simulink model "Porsche930Turbo_Model_V0"  (R2025b)
settings: Solver=ode3  StartTime=0.0  StopTime=1800  FixedStep=0.005  MaxStep=0.01  RelTol=1e-3
values from neighbouring files (symbols this model uses):
  a_front = (1 - CoG_front) * wb    (= 1.32912)    [Main.m]
  af = 1.77    [Main.m]
  bsfc = 395    [Main.m]
  cd = 0.39    [Main.m]
  crr = 0.015    [Main.m]
  distance_imola = s_track    [Main.m]
  eta_gb = 0.95    [Main.m]
  gear_numbers = [1, 2, 3, 4]    [Main.m]
  gear_ratios = [2.25, 1.30, 0.89, 0.625]    [Main.m]
  gear_shift_tbl = [1, 2, 3, 4]    [Main.m]
  grade_imola = grade_track    [Main.m]
  kt = 1.65    [Main.m]
  m_eq = mg + (J_wheels / rw^2) + (J_drivetrain * i_avg^2 / rw^2)    [Main.m]
  mg = mc + (mh * np) + mp_hybrid    (= 1492.5)    [Main.m]
  mu_road = 0.9    [Main.m]
  n_ice = 0:dn:nd    [Main.m]
  ne_em = 0:dn:nemax_em    [Main.m]
  nparallel = 2    [Main.m]
  nseries = 96    [Main.m]
  rho_fuel = 0.75    [Main.m]
  ro = 1.204    [Main.m]
  rt = 4.222    [Main.m]
  rw = (dw * 25.4 / 2 + wt * art / 100) * 1e-3    (= 0.31345)    [Main.m]
  t_ice = zeros(size(n_ice))    [Main.m]
  t_roma_san_basilio = [0 1 2 3 4 5 6 7 8 9 10 11 ... (522 elements, 522x1)]    [ECE_EUDC_Artemis_Bologna_Roma_WLTC_EE_bus.mat]
  tau_turbo = 0.6    [Main.m]
  te_em = zeros(size(ne_em))    [Main.m]
  te_em_peak = zeros(size(ne_em))    [Main.m]
  temax_em = 230    [Main.m]
  tmax_ice = 412    [Main.m]
  track_length = 4909    [Main.m]
  v_cutoff_bp = [0, 0.5, 1.4, 50]    [Main.m]
  v_cutoff_tbl = [0, 0,   1,   1 ]    [Main.m]
  v_ref_imola = v_track_ms    [Main.m]
  v_shift_bp = [0, 18, 33, 48]    [Main.m]
  v_shift_bp_EMODE = [0, 5, 22, 35]    [Main.m]
  vkm_roma_san_basilio = [28.8 30.9 32.4 34.2 35.3 35.6 34.8 33.8 32.2 30.5 29.1 27.9 ... (522 elements, 522x1)]    [ECE_EUDC_Artemis_Bologna_Roma_WLTC_EE_bus.mat]
  wb = 2.272    [Main.m]
undefined symbols (not defined in the file or in its folder): SoC_Per
libraries: simulink x58
(part 4 of 5)

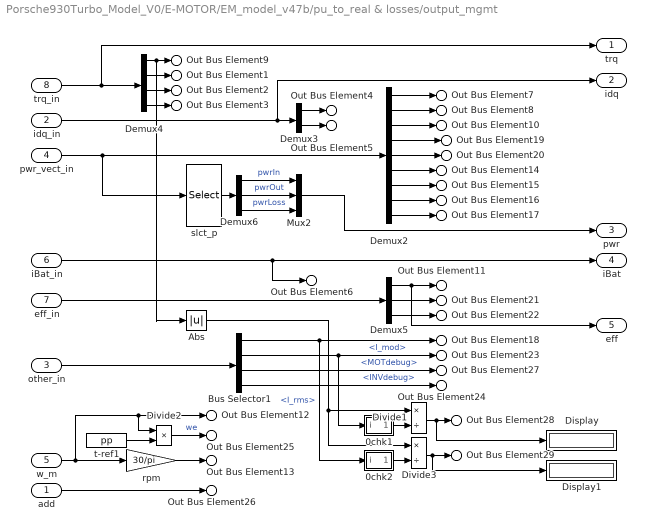
== system Porsche930Turbo_Model_V0/E-MOTOR/EM_model_v47b/pu_to_real & losses/output_mgmt ==
  add : Inport
  idq_in : Inport  Port=2
  other_in : Inport  Port=3
  pwr_vect_in : Inport  Port=4
  w_m : Inport  Port=5
  iBat_in : Inport  Port=6
  eff_in : Inport  Port=7
  trq_in : Inport  Port=8
  0chk1 : Subsystem
      mask Display: disp('0chk')
  0chk2 : Subsystem
      mask Display: disp('0chk')
  Abs : Abs  SaturateOnIntegerOverflow=off
  Bus Selector1 : BusSelector  OutputSignals=I_rms,I_mod,MOTdebug,INVdebug
  Demux2 : Demux  Outputs=9
  Demux3 : Demux  Outputs=2
  Demux4 : Demux
  Demux5 : Demux  Outputs=3
  Demux6 : Demux  Outputs=3
  Display : Display
  Display1 : Display
  Divide1 : Product  Inputs=*/
  Divide2 : Product  Inputs=**
  Divide3 : Product  Inputs=*/
  Mux2 : Mux  Inputs=3
  rpm : Gain  Gain=30/pi  OutDataTypeStr=double
  slct_p : Selector  InputPortWidth=9  IndexOptions=Index vector (dialog)  Indices=[1 2 3]  OutputSizes=1
  t-ref1 : Constant  Value=pp
  trq : Outport
  idq : Outport  Port=2
  pwr : Outport  Port=3
  iBat : Outport  Port=4
  eff : Outport  Port=5
  Out Bus Element9 : Outport  Port=6  PortName=oBus  Element=trqOut
  Out Bus Element1 : Outport  Port=6  PortName=oBus  Element=trqRef
  Out Bus Element2 : Outport  Port=6  PortName=oBus  Element=trqMax
  Out Bus Element3 : Outport  Port=6  PortName=oBus  Element=trqMin
  Out Bus Element4 : Outport  Port=6  PortName=oBus  Element=id
  Out Bus Element5 : Outport  Port=6  PortName=oBus  Element=iq
  Out Bus Element6 : Outport  Port=6  PortName=oBus  Element=iBat
  Out Bus Element18 : Outport  Port=6  PortName=oBus  Element=Irms
  Out Bus Element23 : Outport  Port=6  PortName=oBus  Element=Imod
  Out Bus Element7 : Outport  Port=6  PortName=oBus  Element=pwrIn
  Out Bus Element8 : Outport  Port=6  PortName=oBus  Element=pwrOut
  Out Bus Element10 : Outport  Port=6  PortName=oBus  Element=pwrLoss
  Out Bus Element11 : Outport  Port=6  PortName=oBus  Element=effTot
  Out Bus Element14 : Outport  Port=6  PortName=oBus  Element=pwrOut_Max
  Out Bus Element15 : Outport  Port=6  PortName=oBus  Element=pwrOut_Min
  Out Bus Element16 : Outport  Port=6  PortName=oBus  Element=pwrIn_Max
  Out Bus Element17 : Outport  Port=6  PortName=oBus  Element=pwrIn_Min
  Out Bus Element19 : Outport  Port=6  PortName=oBus  Element=motLosses
  Out Bus Element20 : Outport  Port=6  PortName=oBus  Element=invLosses
  Out Bus Element21 : Outport  Port=6  PortName=oBus  Element=effMot
  Out Bus Element22 : Outport  Port=6  PortName=oBus  Element=effInv
  Out Bus Element28 : Outport  Port=6  PortName=oBus  Element=Kt
  Out Bus Element29 : Outport  Port=6  PortName=oBus  Element=Kt_rms
  Out Bus Element12 : Outport  Port=6  PortName=oBus  Element=w_mec_rads
  Out Bus Element13 : Outport  Port=6  PortName=oBus  Element=w_mec_rpm
  Out Bus Element25 : Outport  Port=6  PortName=oBus  Element=w_ele_rads
  Out Bus Element26 : Outport  Port=6  PortName=oBus  Element=additional
  Out Bus Element24 : Outport  Port=6  PortName=oBus  Element=INVdebug
  Out Bus Element27 : Outport  Port=6  PortName=oBus  Element=MOTdebug
  wires:
  Demux4/1 -> Abs/1, Out Bus Element9/1
  Demux3/1 -> Out Bus Element4/1
  eff_in/1 -> Demux5/1
  Bus Selector1/4 -> Out Bus Element24/1  "<INVdebug>"
  Demux2/6 -> Out Bus Element14/1
  Bus Selector1/2 -> Out Bus Element23/1, 0chk1/1(i)  "<I_mod>"
  Demux2/1 -> Out Bus Element7/1
  Demux4/3 -> Out Bus Element2/1
  Demux3/2 -> Out Bus Element5/1
  Demux2/2 -> Out Bus Element8/1
  Demux5/3 -> Out Bus Element22/1
  Demux2/7 -> Out Bus Element15/1
  Demux2/9 -> Out Bus Element17/1
  Demux4/4 -> Out Bus Element3/1
  Demux4/2 -> Out Bus Element1/1
  Demux2/4 -> Out Bus Element19/1
  Demux2/3 -> Out Bus Element10/1
  Demux2/5 -> Out Bus Element20/1
  Demux5/2 -> Out Bus Element21/1
  Demux2/8 -> Out Bus Element16/1
  Bus Selector1/1 -> Out Bus Element18/1, 0chk2/1(i)  "<I_rms>"
  rpm/1 -> Out Bus Element13/1
  w_m/1 -> Divide2/1, Out Bus Element12/1, rpm/1
  other_in/1 -> Bus Selector1/1
  trq_in/1 -> trq/1, Demux4/1
  slct_p/1 -> Demux6/1
  idq_in/1 -> idq/1, Demux3/1
  pwr_vect_in/1 -> Demux2/1, slct_p/1
  Demux6/3 -> Mux2/3  "pwrLoss"
  Demux6/1 -> Mux2/1  "pwrIn"
  iBat_in/1 -> Out Bus Element6/1, iBat/1
  Mux2/1 -> pwr/1
  Demux5/1 -> Out Bus Element11/1, eff/1
  Demux6/2 -> Mux2/2  "pwrOut"
  t-ref1/1 -> Divide2/2
  Divide2/1 -> Out Bus Element25/1  "we"
  add/1 -> Out Bus Element26/1
  Bus Selector1/3 -> Out Bus Element27/1  "<MOTdebug>"
  Divide1/1 -> Display/1, Out Bus Element28/1
  Divide3/1 -> Out Bus Element29/1, Display1/1
  0chk2/1(o) -> Divide3/2
  0chk1/1(o) -> Divide1/2
  Abs/1 -> Divide3/1, Divide1/1

== system Porsche930Turbo_Model_V0/E-MOTOR/EM_model_v47b/pu_to_real & losses/pwr_calc ==
  pwr_loss : Inport
  w_m : Inport  Port=2
  trq : Inport  Port=3
  Demux4 : Demux  Outputs=2
  Divide2 : Product  Inputs=**
  Divide3 : Product  Inputs=**
  MaxMin : Selector  InputPortWidth=4  IndexOptions=Index vector (dialog)  Indices=[3 4]  OutputSizes=1
  Mux5 : Mux  Inputs=7
  Sum1 : Sum
  Sum2 : Sum
  Sum3 : Sum  Inputs=+
  trq_out : Selector  InputPortWidth=4  IndexOptions=Index vector (dialog)  Indices=1  OutputSizes=1
  pwr_vect : Outport
  pwrIN : Outport  Port=2
  wires:
  w_m/1 -> Divide3/1, Divide2/1
  trq_out/1 -> Divide2/2
  trq/1 -> trq_out/1, MaxMin/1
  MaxMin/1 -> Divide3/2
  Divide3/1 -> Sum2/1, Mux5/6  "pwrMaxOUT"
  Sum2/1 -> Mux5/7  "pwrMaxIN"
  Sum3/1 -> Mux5/3, Sum2/2, Sum1/1  "pwrLOSS"
  Divide2/1 -> Sum1/2, Mux5/2  "pwrOUT"
  Sum1/1 -> pwrIN/1, Mux5/1  "pwrIN"
  Mux5/1 -> pwr_vect/1
  pwr_loss/1 -> Demux4/1, Sum3/1
  Demux4/1 -> Mux5/4  "mot_loss"
  Demux4/2 -> Mux5/5  "inv_loss"

== system Porsche930Turbo_Model_V0/E-MOTOR/EM_model_v47b/pu_to_real & losses/trq_derating_TBD ==
  note: recalculation of Irms
      | saturated, mainly for
      | verification
  note: linear idq is increased
      | by "saturation coeff"
  note: outputs Irms saturated
      | given the torque input
  note: VERIFICATION
  idq : Inport
  idq_pu : Inport  Port=2
  trq_pu : Inport  Port=3
  trqIn : Inport  Port=4
  0chk : Subsystem
      mask Display: disp('0chk')
  0chk1 : Subsystem
      mask Display: disp('0chk')
  0chk2 : Subsystem
      mask Display: disp('0chk')
  Abs1 : Abs  SaturateOnIntegerOverflow=off
  DQmodule : Subsystem
      mask Display: disp('DQmod')
  DQmodule1 : Subsystem
      mask Display: disp('DQmod')
  DQmodule2 : Subsystem
      mask Display: disp('DQmod')
  Divide1 : Product  Inputs=**
  Divide2 : Product  Inputs=*/
  Divide4 : Product  Inputs=/*
  Divide5 : Product  Inputs=/*
  peak2rms : Subsystem
      mask Display: disp('pk2rms')
  peak2rms1 : Subsystem
      mask Display: disp('pk2rms')
  peak2rms2 : Subsystem
      mask Display: disp('pk2rms')
  sc{1..3,5,8} (5 alike) : Scope  NumInputPorts=2
      sc1 settings: DataLoggingSaveFormat=Array
      sc2 settings: DataLoggingVariableName=ScopeData5  DataLoggingSaveFormat=Array
      sc3 settings: DataLoggingVariableName=ScopeData5  DataLoggingSaveFormat=Array
      sc5 settings: DataLoggingVariableName=ScopeData9  DataLoggingSaveFormat=Array
      sc8 settings: DataLoggingVariableName=ScopeData13  DataLoggingSaveFormat=Array
  sc6 : Scope  NumInputPorts=3
      settings: DataLoggingVariableName=ScopeData10  DataLoggingSaveFormat=Array
  trq vs curr : Lookup_n-D  NumberOfTableDimensions=1  BreakpointsForDimension1=[0 0.5 0.75 1 1.4 1.8 2.5 3]  BeginIndexSearchUsingPreviousIndexResult=on  Table=[0 0.5 0.75 1 1.5 2 3 4]  InternalRulePriority=Speed  RndMeth=Simplest
  trq_out : Selector  InputPortWidth=4  IndexOptions=Index vector (dialog)  Indices=1  OutputSizes=1
  trq_outPU : Selector  InputPortWidth=4  IndexOptions=Index vector (dialog)  Indices=1  OutputSizes=1
  idq_sat : Outport
  wires:
  trqIn/1 -> trq_out/1
  trq_out/1 -> Divide5/2, Divide4/2
  peak2rms1/1(o) -> 0chk1/1(i)
  trq vs curr/1 -> sc2/2, sc6/2, Divide2/1  "Irms"
  idq/1 -> Divide1/1, DQmodule1/1(i), sc1/1
  Divide2/1 -> sc3/2, Divide1/2
  Divide1/1 -> DQmodule2/1(i), idq_sat/1
  peak2rms2/1(o) -> 0chk2/1(i), sc6/1
  Divide4/1 -> sc8/2
  Divide5/1 -> sc8/1
  DQmodule1/1(mod) -> peak2rms1/1(i), sc5/1, sc1/2
  0chk1/1(o) -> sc2/1, Divide4/1, sc6/3
  0chk2/1(o) -> Divide5/1
  idq_pu/1 -> DQmodule/1(i)
  trq_pu/1 -> trq_outPU/1
  trq_outPU/1 -> Abs1/1
  peak2rms/1(o) -> 0chk/1(i)
  DQmodule/1(mod) -> peak2rms/1(i)
  0chk/1(o) -> sc3/1, Divide2/2
  Abs1/1 -> trq vs curr/1
  DQmodule2/1(mod) -> peak2rms2/1(i), sc5/2

== system Porsche930Turbo_Model_V0/E-MOTOR/EM_model_v47b/real_to_pu & param/input_iLim ==
  i : Inport
  Display1 : Display
  Multiport Switch1 : MultiPortSwitch  SaturateOnIntegerOverflow=off  InputSameDT=off
  t-ref2 : Constant  Value=overl
  t-ref7 : Constant  Value=i_lim
  t-ref8 : Constant
  iLim : Outport
  wires:
  i/1 -> Multiport Switch1/4  "from port"
  Multiport Switch1/1 -> iLim/1
  t-ref2/1 -> Display1/1, Multiport Switch1/1
  t-ref7/1 -> Multiport Switch1/3  "static"
  t-ref8/1 -> Multiport Switch1/2  "no overload"

== system Porsche930Turbo_Model_V0/E-MOTOR/EM_model_v47b/real_to_pu & param/input_rs ==
  i : Inport
  Display6 : Display
  Multiport Switch1 : MultiPortSwitch  SaturateOnIntegerOverflow=off  InputSameDT=off
  n 1 : Constant  Value=rs
  n 2 : Constant  Value=1e-6
  t-ref1 : Constant  Value=RsSlct
  rs : Outport
  wires:
  i/1 -> Multiport Switch1/4  "from port"
  Multiport Switch1/1 -> rs/1
  t-ref1/1 -> Multiport Switch1/1, Display6/1
  n 2/1 -> Multiport Switch1/2  "no stator res"
  n 1/1 -> Multiport Switch1/3  "static"

== system Porsche930Turbo_Model_V0/E-MOTOR/EM_model_v47b/real_to_pu & param/input_spd ==
  i : Inport
  Display1 : Display
  Multiport Switch1 : MultiPortSwitch  Inputs=2  SaturateOnIntegerOverflow=off  InputSameDT=off
  rad/s : Gain  Gain=pi/30  OutDataTypeStr=double
  t-ref : Constant  Value=spdIn
  rads : Outport
  wires:
  rad/s/1 -> Multiport Switch1/2
  i/1 -> rad/s/1, Multiport Switch1/3
  Multiport Switch1/1 -> rads/1
  t-ref/1 -> Multiport Switch1/1, Display1/1

== system Porsche930Turbo_Model_V0/E-MOTOR/EM_model_v47b/real_to_pu & param/spd_0chk ==
  i : Inport
  Abs : Abs  SaturateOnIntegerOverflow=off
  MinMax1 : MinMax  Function=max  Inputs=2
  Switch3 : Switch  SaturateOnIntegerOverflow=off  InputSameDT=off
  V1 : Constant  Value=-1
  V3 : Constant
  n 2 : Constant  Value=1e-4
  x1 : Product  Inputs=**
  o : Outport
  wires:
  n 2/1 -> MinMax1/2
  Switch3/1 -> x1/1
  i/1 -> Switch3/2, Abs/1
  Abs/1 -> MinMax1/1
  x1/1 -> o/1
  V3/1 -> Switch3/1
  V1/1 -> Switch3/3
  MinMax1/1 -> x1/2

== system Porsche930Turbo_Model_V0/E-MOTOR/EM_model_v47b/real_to_pu & param/trq_0chk ==
  i : Inport
  Abs1 : Abs  SaturateOnIntegerOverflow=off
  MinMax1 : MinMax  Function=max  Inputs=2
  Relational Operator1 : RelationalOperator  Operator=<  OutDataTypeStr=boolean  InputSameDT=off
  Switch1 : Switch  SaturateOnIntegerOverflow=off  InputSameDT=off
  V2 : Constant  Value=-1
  V4 : Constant
  range : Constant  Value=0.01
  x1 : Product  Inputs=**
  ctrl0 : Outport
  "o " : Outport  Port=2
  wires:
  x1/1 -> "o "/1
  MinMax1/1 -> x1/2
  V2/1 -> Switch1/3
  V4/1 -> Switch1/1
  Abs1/1 -> Relational Operator1/1, MinMax1/1
  i/1 -> Switch1/2, Abs1/1
  Switch1/1 -> x1/1
  range/1 -> Relational Operator1/2, MinMax1/2
  Relational Operator1/1 -> ctrl0/1

== system Porsche930Turbo_Model_V0/Battery Pack/Subsystem/Thermal Model/Subsystem/Subsystem ==
  R1 [°C/W] : Inport
  R2 [°C/W] : Inport  Port=2
  R3 [°C/W] : Inport  Port=3
  C1 [J/°C] : Inport  Port=4
  C2 [J/°C] : Inport  Port=5
  Sum : Sum
  Tau : Sum  Inputs=+++
  Tau1 : Product
  Tau12 : Product
  Tau2 : Product
  tau [J/W] : Outport
  tau1 [J/W] : Outport  Port=2
  tau2 [J/W] : Outport  Port=3
  tau12 [J/W] : Outport  Port=4
  wires:
  Tau1/1 -> tau1 [J/W]/1, Tau/1
  Sum/1 -> Tau12/1, Tau2/1
  Tau2/1 -> Tau/2, tau2 [J/W]/1
  C2 [J/°C]/1 -> Tau2/2
  Tau12/1 -> Tau/3, tau12 [J/W]/1
  Tau/1 -> tau [J/W]/1
  C1 [J/°C]/1 -> Tau1/2, Tau12/2
  R1 [°C/W]/1 -> Tau1/1
  R3 [°C/W]/1 -> Sum/2
  R2 [°C/W]/1 -> Sum/1

== system Porsche930Turbo_Model_V0/Battery Pack/Subsystem/Thermal Model/Subsystem1/Subsystem ==
  R1 [°C/W] : Inport
  R3 [°C/W] : Inport  Port=2
  C1 [J/°C] : Inport  Port=3
  Product : Product
  Sum : Sum
  tau [J/W] : Outport
  wires:
  R3 [°C/W]/1 -> Sum/2
  R1 [°C/W]/1 -> Sum/1
  Sum/1 -> Product/1
  C1 [J/°C]/1 -> Product/2
  Product/1 -> tau [J/W]/1

== system Porsche930Turbo_Model_V0/E-MOTOR/EM_model_v47b/Motor_Model/blockB/module MTV ==
  i : Inport
  Add : Sum
  Demux2 : Demux  Outputs=2
  Product : Product
  Product1 : Product
  Sqrt : Sqrt
  mod : Outport
  wires:
  Demux2/1 -> Product/2, Product/1
  Sqrt/1 -> mod/1
  Product/1 -> Add/1
  Demux2/2 -> Product1/1, Product1/2
  Add/1 -> Sqrt/1
  Product1/1 -> Add/2
  i/1 -> Demux2/1

== system Porsche930Turbo_Model_V0/E-MOTOR/EM_model_v47b/Motor_Model/blockB/module TF ==
  i : Inport
  Add : Sum
  Demux2 : Demux  Outputs=2
  Product : Product
  Product1 : Product
  Sqrt : Sqrt
  mod : Outport
  wires:
  Demux2/1 -> Product/2, Product/1
  Sqrt/1 -> mod/1
  Product/1 -> Add/1
  Demux2/2 -> Product1/1, Product1/2
  Add/1 -> Sqrt/1
  Product1/1 -> Add/2
  i/1 -> Demux2/1

== system Porsche930Turbo_Model_V0/E-MOTOR/EM_model_v47b/Motor_Model/blockC/0chk ==
  i : Inport
  Abs : Abs  SaturateOnIntegerOverflow=off
  MinMax1 : MinMax  Function=max  Inputs=2
  Switch3 : Switch  SaturateOnIntegerOverflow=off  InputSameDT=off
  V1 : Constant  Value=-1
  V3 : Constant
  n 2 : Constant  Value=1e-6
  x1 : Product  Inputs=**
  o : Outport
  wires:
  n 2/1 -> MinMax1/2
  Switch3/1 -> x1/1
  i/1 -> Switch3/2, Abs/1
  Abs/1 -> MinMax1/1
  x1/1 -> o/1
  V3/1 -> Switch3/1
  V1/1 -> Switch3/3
  MinMax1/1 -> x1/2

== system Porsche930Turbo_Model_V0/E-MOTOR/EM_model_v47b/Motor_Model/blockD/idq_max_MTC-I0 ==
  trq : Inport
  I0 : Inport  Port=2
  "0 " : Constant  Value=0
  Compare To Constant3 : simulink/Logic and Bit Operations/Compare To Constant  relop===  const=1  OutDataTypeStr=boolean
  Constant4 : Constant  Value=r
  Divide2 : Product  Inputs=**
  Gain1 : Gain  Gain=-1
  Mux2 : Mux  Inputs=2
  Mux5 : Mux  Inputs=2
  Switch7 : Switch  Criteria=u2 > Threshold  SaturateOnIntegerOverflow=off  InputSameDT=off
  id_mtcMax : Subsystem
  iq_mtcMax : Subsystem
  sign : Subsystem
  idq_mtcMaxPos : Outport
  idq_mtcMaxNeg : Outport  Port=2
  wires:
  Switch7/1 -> iq_mtcMax/2(id), Mux5/1, Mux2/1
  "0 "/1 -> Switch7/1
  I0/1 -> iq_mtcMax/1(IO), id_mtcMax/1(I0)
  sign/1(o) -> Divide2/2
  trq/1 -> sign/1(i)
  Constant4/1 -> Compare To Constant3/1
  Compare To Constant3/1 -> Switch7/2
  iq_mtcMax/1(iq) -> Divide2/1
  id_mtcMax/1(id_MTC) -> Switch7/3
  Divide2/1 -> Gain1/1, Mux5/2
  Mux5/1 -> idq_mtcMaxPos/1
  Gain1/1 -> Mux2/2
  Mux2/1 -> idq_mtcMaxNeg/1

== system Porsche930Turbo_Model_V0/E-MOTOR/EM_model_v47b/Motor_Model/blockD/idq_max_MTV-I0 ==
  b : Inport
  theta : Inport  Port=2
  trq : Inport  Port=3
  I0 : Inport  Port=4
  Gain2 : Gain  Gain=-1
  Mux1 : Mux  Inputs=2
  Mux3 : Mux  Inputs=2
  a : Constant  Value=a
  intersections_neg : MATLAB Function  TreatAsAtomicUnit=on
  intersections_pos : MATLAB Function  TreatAsAtomicUnit=on
  r 1 : Constant  Value=r
  sc1 : Scope  NumInputPorts=2
      settings: DataLoggingVariableName=ScopeData5  DataLoggingSaveFormat=Array
  sc2 : Scope  NumInputPorts=2
      settings: DataLoggingVariableName=ScopeData4  DataLoggingSaveFormat=Array
  flg_maxSpd : Outport
  idq_mtvMaxPos : Outport  Port=2
  idq_mtvMaxNeg : Outport  Port=3
  wires:
  a/1 -> intersections_neg/1(a), intersections_pos/1(a)
  r 1/1 -> intersections_neg/2(r), intersections_pos/2(r)
  intersections_pos/1(id) -> Mux3/1  "id_mtv"
  intersections_pos/2(iq) -> Mux3/2  "iq_mtv"
  intersections_pos/3(discr) -> sc2/2, flg_maxSpd/1
  b/1 -> intersections_neg/3(b), intersections_pos/3(b)
  I0/1 -> intersections_neg/4(I0), intersections_pos/4(I0)
  theta/1 -> intersections_neg/5(theta), intersections_pos/5(theta)
  trq/1 -> Gain2/1, intersections_pos/6(t)
  Gain2/1 -> intersections_neg/6(t)
  intersections_neg/1(id) -> Mux1/1  "id_mtv"
  intersections_neg/2(iq) -> Mux1/2  "iq_mtv"
  Mux3/1 -> sc2/1, idq_mtvMaxPos/1
  Mux1/1 -> sc1/1, idq_mtvMaxNeg/1
  intersections_neg/3(discr) -> sc1/2

== system Porsche930Turbo_Model_V0/E-MOTOR/EM_model_v47b/Motor_Model/blockD/iso controller ==
  id_b_pos : Inport
  id_b_neg : Inport  Port=2
  id_MTC : Inport  Port=3
  Compare To Constant : simulink/Logic and Bit Operations/Compare To Constant  relop=>  const=1  OutDataTypeStr=boolean
  Compare To Constant1 : simulink/Logic and Bit Operations/Compare To Constant  relop=~=  const=0  OutDataTypeStr=boolean
  Compare To Constant2 : simulink/Logic and Bit Operations/Compare To Constant  relop=~=  const=0  OutDataTypeStr=boolean
  Compare To Constant3 : simulink/Logic and Bit Operations/Compare To Constant  relop===  const=1  OutDataTypeStr=boolean
  Constant : Constant  Value=r
  Constant4 : Constant  Value=r
  Constant5 : Constant  Value=0
  Logical Operator : Logic  AllPortsSameDT=off  OutDataTypeStr=boolean
  Logical Operator1 : Logic  AllPortsSameDT=off  OutDataTypeStr=boolean
  Relational Operator1 : RelationalOperator  Operator=<=  OutDataTypeStr=boolean  InputSameDT=off
  Relational Operator3 : RelationalOperator  Operator=<=  OutDataTypeStr=boolean  InputSameDT=off
  Switch1 : Switch  Criteria=u2 > Threshold  SaturateOnIntegerOverflow=off  InputSameDT=off
  Switch2 : Switch  Criteria=u2 > Threshold  SaturateOnIntegerOverflow=off  InputSameDT=off
  Switch3 : Switch  Criteria=u2 > Threshold  SaturateOnIntegerOverflow=off  InputSameDT=off
  scope2 : Scope  NumInputPorts=2
      settings: DataLoggingSaveFormat=Array
  cont_pos : Outport
  cont_neg : Outport  Port=2
  wires:
  Constant/1 -> Compare To Constant/1
  Switch2/1 -> scope2/1, cont_pos/1
  Compare To Constant/1 -> Switch1/2, Switch2/2
  Relational Operator3/1 -> Switch2/3, Logical Operator/1
  Compare To Constant1/1 -> Logical Operator/2
  Logical Operator/1 -> Switch2/1
  id_b_pos/1 -> Compare To Constant1/1, Relational Operator3/1
  Switch3/1 -> Relational Operator3/2, Relational Operator1/2
  id_MTC/1 -> Switch3/3
  Constant4/1 -> Compare To Constant3/1
  Compare To Constant3/1 -> Switch3/2
  Constant5/1 -> Switch3/1
  Compare To Constant2/1 -> Logical Operator1/2
  Relational Operator1/1 -> Switch1/3, Logical Operator1/1
  Logical Operator1/1 -> Switch1/1
  id_b_neg/1 -> Compare To Constant2/1, Relational Operator1/1
  Switch1/1 -> scope2/2, cont_neg/1

== system Porsche930Turbo_Model_V0/E-MOTOR/EM_model_v47b/Motor_Model/blockE/module ==
  in : Inport
  Add : Sum
  Demux2 : Demux  Outputs=2
  Product : Product
  Product1 : Product
  Sqrt : Sqrt
  module : Outport
  wires:
  Demux2/1 -> Product/2, Product/1
  Sqrt/1 -> module/1
  Product/1 -> Add/1
  Demux2/2 -> Product1/1, Product1/2
  Add/1 -> Sqrt/1
  Product1/1 -> Add/2
  in/1 -> Demux2/1

== system Porsche930Turbo_Model_V0/E-MOTOR/EM_model_v47b/Motor_Model/limit_rpm/trq calc ==
  idq : Inport
  Add : Sum
  Constant10 : Constant  Value=r1
  Constant11 : Constant  Value=a
  Demux1 : Demux  Outputs=2
  Product3 : Product  Inputs=3
  Product7 : Product
  trq : Outport
  wires:
  idq/1 -> Demux1/1
  Constant10/1 -> Product3/3
  Add/1 -> trq/1
  Demux1/1 -> Product3/1
  Product7/1 -> Add/2
  Product3/1 -> Add/1
  Demux1/2 -> Product7/1, Product3/2
  Constant11/1 -> Product7/2

== system Porsche930Turbo_Model_V0/E-MOTOR/EM_model_v47b/Motor_Model/limits_MaxMin/DQmodule ==
  i : Inport
  Add : Sum
  Demux2 : Demux  Outputs=2
  Product : Product
  Product1 : Product
  Sqrt : Sqrt
  mod : Outport
  wires:
  Demux2/1 -> Product/2, Product/1
  Sqrt/1 -> mod/1
  Product/1 -> Add/1
  Demux2/2 -> Product1/1, Product1/2
  Add/1 -> Sqrt/1
  Product1/1 -> Add/2
  i/1 -> Demux2/1

== system Porsche930Turbo_Model_V0/E-MOTOR/EM_model_v47b/Motor_Model/limits_MaxMin/MTV_sat_low spd ==
  i_lim : Inport
  idq_ref : Inport  Port=2
  mod_chk : Inport  Port=3
  Demux2 : Demux
  Demux6 : Demux  Outputs=2
  MinMax3 : MinMax  Function=max  Inputs=2
  MinMax4 : MinMax  Inputs=2
  MinMax5 : MinMax  Function=max  Inputs=2
  MinMax6 : MinMax  Inputs=2
  Mux14 : Mux  Inputs=2
  SatDyn : simulink/Discontinuities/Saturation Dynamic  OutMin=[]  OutMax=[]  OutDataTypeStr=Inherit: Same as second input  OutDataType=fixdt(1, 16)  OutScaling=2^-10  DoSatur=off
  SatDyn1 : simulink/Discontinuities/Saturation Dynamic  OutMin=[]  OutMax=[]  OutDataTypeStr=Inherit: Same as second input  OutDataType=fixdt(1, 16)  OutScaling=2^-10  DoSatur=off
  Switch12 : Switch  Criteria=u2 > Threshold  SaturateOnIntegerOverflow=off  InputSameDT=off
  idq_sat : Outport
  wires:
  Mux14/1 -> Switch12/1
  Demux6/2 -> SatDyn1/2  "iq"
  mod_chk/1 -> Switch12/2
  Demux6/1 -> SatDyn/2  "id"
  MinMax6/1 -> SatDyn1/3
  MinMax3/1 -> SatDyn/1
  MinMax4/1 -> SatDyn/3
  Demux2/3 -> MinMax3/2, MinMax4/2  "id2"
  Demux2/2 -> MinMax5/1, MinMax6/1  "iq1"
  Demux2/4 -> MinMax6/2, MinMax5/2  "iq2"
  Demux2/1 -> MinMax4/1, MinMax3/1  "id1"
  MinMax5/1 -> SatDyn1/1
  Switch12/1 -> idq_sat/1
  SatDyn1/1 -> Mux14/2
  SatDyn/1 -> Mux14/1
  idq_ref/1 -> Demux6/1, Switch12/3
  i_lim/1 -> Demux2/1

== system Porsche930Turbo_Model_V0/E-MOTOR/EM_model_v47b/Motor_Model/limits_MaxMin/current limits calc ==
  I0 : Inport
  I0_lim : Inport  Port=2
  MTV_lim : Inport  Port=3
  Comp2Const2 : simulink/Logic and Bit Operations/Compare To Constant  relop===  const=0  OutDataTypeStr=boolean
  Comp2Const3 : simulink/Logic and Bit Operations/Compare To Constant  relop===  const=0  OutDataTypeStr=boolean
  DQmodule : Subsystem
      mask Display: disp('DQmod')
  DQmodule1 : Subsystem
      mask Display: disp('DQmod')
  Demux1 : Demux
  Demux4 : Demux
  Logical Operator3 : Logic  Operator=OR  AllPortsSameDT=off  OutDataTypeStr=boolean
  Logical Operator4 : Logic  Operator=OR  AllPortsSameDT=off  OutDataTypeStr=boolean
  Mux{2..3,5..6,8} (5 alike) : Mux  Inputs=2
  Relational Operator1 : RelationalOperator  Operator=>  OutDataTypeStr=boolean  InputSameDT=off
  Relational Operator3 : RelationalOperator  Operator=>  OutDataTypeStr=boolean  InputSameDT=off
  Switch3 : Switch  Criteria=u2 > Threshold  SaturateOnIntegerOverflow=off  InputSameDT=off
  Switch6 : Switch  Criteria=u2 > Threshold  SaturateOnIntegerOverflow=off  InputSameDT=off
  losses4 : Scope  NumInputPorts=2
      settings: DataLoggingVariableName=ScopeData12  DataLoggingSaveFormat=Array
  losses6 : Scope  NumInputPorts=3
      settings: DataLoggingVariableName=ScopeData15  DataLoggingSaveFormat=Array
  i_limit_MaxMin : Outport
  moduleMTV : Outport  Port=2
  wires:
  MTV_lim/1 -> Demux4/1
  Mux3/1 -> [I0_lim2]
  Relational Operator3/1 -> Logical Operator4/1
  Relational Operator1/1 -> Logical Operator3/1
  Demux1/4 -> Mux3/2
  Demux4/4 -> Mux2/2
  Switch3/1 -> Mux8/1
  Demux1/1 -> Mux6/1
  Demux4/1 -> Mux5/1
  Demux1/2 -> Mux6/2
  Mux6/1 -> [I0_lim1]
  Switch6/1 -> Mux8/2
  Comp2Const3/1 -> Logical Operator4/2
  I0/1 -> losses6/3, Relational Operator3/2, Relational Operator1/2
  Mux8/1 -> i_limit_MaxMin/1
  Comp2Const2/1 -> Logical Operator3/2
  Logical Operator3/1 -> Switch3/2, losses4/1
  DQmodule/1(mod) -> losses6/2, moduleMTV/1, Comp2Const3/1, Relational Operator3/1
  Demux1/3 -> Mux3/1
  Mux5/1 -> DQmodule1/1(i), [mtv_lim1]
  Logical Operator4/1 -> Switch6/2, losses4/2
  Demux4/2 -> Mux5/2
  DQmodule1/1(mod) -> Relational Operator1/1, Comp2Const2/1, losses6/1
  I0_lim/1 -> Demux1/1
  Demux4/3 -> Mux2/1
  Mux2/1 -> DQmodule/1(i), [mtv_lim2]
  [I0_lim1] -> Switch3/1
  [I0_lim2] -> Switch6/1
  [mtv_lim1] -> Switch3/3
  [mtv_lim2] -> Switch6/3

== system Porsche930Turbo_Model_V0/E-MOTOR/EM_model_v47b/Motor_Model/limits_MaxMin/iq from trq+idsat ==
  trq : Inport
  Add1 : Sum
  Constant10 : Constant  Value=r1
  Constant4 : Constant  Value=a
  Constant5 : Constant  Value=sat
  Product1 : Product
  Product2 : Product  Inputs=*/
  scope1 : Scope  NumInputPorts=2
      settings: DataLoggingVariableName=ScopeData3  DataLoggingSaveFormat=Array
  iq : Outport
  wires:
  Constant10/1 -> Product1/1
  Constant5/1 -> Product1/2
  Product1/1 -> Add1/1
  Constant4/1 -> Add1/2
  Add1/1 -> Product2/2, scope1/2
  trq/1 -> scope1/1, Product2/1
  Product2/1 -> iq/1

== system Porsche930Turbo_Model_V0/E-MOTOR/EM_model_v47b/Motor_Model/limits_MaxMin/trq calc1 ==
  idq : Inport
  Add : Sum
  Constant10 : Constant  Value=r1
  Constant11 : Constant  Value=a
  Demux1 : Demux  Outputs=2
  Product3 : Product  Inputs=3
  Product7 : Product
  trq : Outport
  wires:
  idq/1 -> Demux1/1
  Constant10/1 -> Product3/3
  Add/1 -> trq/1
  Demux1/1 -> Product3/1
  Product7/1 -> Add/2
  Product3/1 -> Add/1
  Demux1/2 -> Product7/1, Product3/2
  Constant11/1 -> Product7/2

== system Porsche930Turbo_Model_V0/E-MOTOR/EM_model_v47b/Motor_Model/limits_MaxMin/trq calc2 ==
  idq : Inport
  Add : Sum
  Constant10 : Constant  Value=r1
  Constant11 : Constant  Value=a
  Demux1 : Demux  Outputs=2
  Product3 : Product  Inputs=3
  Product7 : Product
  trq : Outport
  wires:
  idq/1 -> Demux1/1
  Constant10/1 -> Product3/3
  Add/1 -> trq/1
  Demux1/1 -> Product3/1
  Product7/1 -> Add/2
  Product3/1 -> Add/1
  Demux1/2 -> Product7/1, Product3/2
  Constant11/1 -> Product7/2

== system Porsche930Turbo_Model_V0/E-MOTOR/EM_model_v47b/Motor_Model/limits_MaxMin/trq calc3 ==
  idq : Inport
  Add : Sum
  Constant10 : Constant  Value=r1
  Constant11 : Constant  Value=a
  Demux1 : Demux  Outputs=2
  Product3 : Product  Inputs=3
  Product7 : Product
  trq : Outport
  wires:
  idq/1 -> Demux1/1
  Constant10/1 -> Product3/3
  Add/1 -> trq/1
  Demux1/1 -> Product3/1
  Product7/1 -> Add/2
  Product3/1 -> Add/1
  Demux1/2 -> Product7/1, Product3/2
  Constant11/1 -> Product7/2

== system Porsche930Turbo_Model_V0/E-MOTOR/EM_model_v47b/pu_to_real & losses/Additional Calc/0chk ==
  i : Inport
  Abs : Abs  SaturateOnIntegerOverflow=off
  MinMax1 : MinMax  Function=max  Inputs=2
  Switch3 : Switch  SaturateOnIntegerOverflow=off  InputSameDT=off
  V1 : Constant  Value=-1
  V3 : Constant
  n 2 : Constant  Value=1e-8
  x1 : Product  Inputs=**
  o : Outport
  wires:
  n 2/1 -> MinMax1/2
  Switch3/1 -> x1/1
  i/1 -> Switch3/2, Abs/1
  Abs/1 -> MinMax1/1
  x1/1 -> o/1
  V3/1 -> Switch3/1
  V1/1 -> Switch3/3
  MinMax1/1 -> x1/2

== system Porsche930Turbo_Model_V0/E-MOTOR/EM_model_v47b/pu_to_real & losses/Additional Calc/0chk1 ==
  i : Inport
  Abs : Abs  SaturateOnIntegerOverflow=off
  MinMax1 : MinMax  Function=max  Inputs=2
  Switch3 : Switch  SaturateOnIntegerOverflow=off  InputSameDT=off
  V1 : Constant  Value=-1
  V3 : Constant
  n 2 : Constant  Value=1e-8
  x1 : Product  Inputs=**
  o : Outport
  wires:
  n 2/1 -> MinMax1/2
  Switch3/1 -> x1/1
  i/1 -> Switch3/2, Abs/1
  Abs/1 -> MinMax1/1
  x1/1 -> o/1
  V3/1 -> Switch3/1
  V1/1 -> Switch3/3
  MinMax1/1 -> x1/2

== system Porsche930Turbo_Model_V0/E-MOTOR/EM_model_v47b/pu_to_real & losses/Additional Calc/DQmodule ==
  i : Inport
  Add : Sum
  Demux2 : Demux  Outputs=2
  Product : Product
  Product1 : Product
  Sqrt : Sqrt
  mod : Outport
  wires:
  Demux2/1 -> Product/2, Product/1
  Sqrt/1 -> mod/1
  Product/1 -> Add/1
  Demux2/2 -> Product1/1, Product1/2
  Add/1 -> Sqrt/1
  Product1/1 -> Add/2
  i/1 -> Demux2/1

== system Porsche930Turbo_Model_V0/E-MOTOR/EM_model_v47b/pu_to_real & losses/Additional Calc/DQmodule1 ==
  i : Inport
  Add : Sum
  Demux2 : Demux  Outputs=2
  Product : Product
  Product1 : Product
  Sqrt : Sqrt
  mod : Outport
  wires:
  Demux2/1 -> Product/2, Product/1
  Sqrt/1 -> mod/1
  Product/1 -> Add/1
  Demux2/2 -> Product1/1, Product1/2
  Add/1 -> Sqrt/1
  Product1/1 -> Add/2
  i/1 -> Demux2/1

== system Porsche930Turbo_Model_V0/E-MOTOR/EM_model_v47b/pu_to_real & losses/Additional Calc/Torque ==
  fiPM : Inport
  idq : Inport  Port=2
  (Ld-Lq)idiq : Product  Inputs=3
  Constant4 : Constant  Value=Lq
  Constant5 : Constant  Value=(3/2)*pp
  Constant6 : Constant  Value=Ld
  Demux2 : Demux  Outputs=2
  Product7 : Product
  Subtract4 : Sum  Inputs=+-
  Subtract5 : Sum
  fiPM*iq : Product
  EM torque : Outport
  wires:
  idq/1 -> Demux2/1
  fiPM/1 -> fiPM*iq/2
  Product7/1 -> EM torque/1  "EM torque"
  Subtract4/1 -> (Ld-Lq)idiq/1  "Ld-Lq"
  Constant6/1 -> Subtract4/1
  Demux2/1 -> (Ld-Lq)idiq/3  "id"
  Constant5/1 -> Product7/1
  Demux2/2 -> fiPM*iq/1, (Ld-Lq)idiq/2  "iq"
  Constant4/1 -> Subtract4/2
  fiPM*iq/1 -> Subtract5/1
  Subtract5/1 -> Product7/2
  (Ld-Lq)idiq/1 -> Subtract5/2

== system Porsche930Turbo_Model_V0/E-MOTOR/EM_model_v47b/pu_to_real & losses/Additional Calc/Voltages ==
  note: % vd = rs*id - w*Lq*iq
      | % vq = rs*iq + w*Ld*id + w*fpm ---> w*PhiPM
  rs : Inport
  idq [A] : Inport  Port=2
  w_e : Inport  Port=3
  Constant : Constant  Value=Ld
  Constant1 : Constant  Value=Lq
  Constant2 : Constant  Value=a
  Constant3 : Constant  Value=Ld
  Constant7 : Constant  Value=In
  Demux : Demux  Outputs=2
  Product{,1..2,5} (4 alike) : Product
  Product3 : Product  Inputs=3
  Product4 : Product  Inputs=3
  Subtract : Sum
  Subtract1 : Sum  Inputs=+-
  Subtract2 : Sum
  vd : Outport
  vq : Outport  Port=2
  fiPM : Outport  Port=3
  wires:
  Demux/1 -> Product1/2, Product2/1  "id"
  Subtract1/1 -> vd/1  "vd"
  Constant/1 -> Product2/2
  Product5/1 -> Subtract/2  "w(Ldid+fiPM)"
  Product3/1 -> Subtract1/2  "wLqiq"
  Constant7/1 -> Product4/3
  w_e/1 -> Product5/2, Product3/3
  Constant2/1 -> Product4/1
  rs/1 -> Product1/1, Product/1
  Demux/2 -> Product/2, Product3/1  "iq"
  Product/1 -> Subtract/1  "Rsiq"
  Product1/1 -> Subtract1/1  "Rsid"
  Subtract/1 -> vq/1  "vq"
  Constant1/1 -> Product3/2
  Product2/1 -> Subtract2/1  "Ldid"
  idq [A]/1 -> Demux/1
  Subtract2/1 -> Product5/1  "(Ldid+fiPM)"
  Product4/1 -> fiPM/1, Subtract2/2  "fiPM"
  Constant3/1 -> Product4/2

== system Porsche930Turbo_Model_V0/E-MOTOR/EM_model_v47b/pu_to_real & losses/Additional Calc/peak2rms ==
  i : Inport
  1/sqrt(2) : Gain  Gain=0.707106781186547
  o : Outport
  wires:
  i/1 -> 1/sqrt(2)/1  "peak value"
  1/sqrt(2)/1 -> o/1  "RMS value"

== system Porsche930Turbo_Model_V0/E-MOTOR/EM_model_v47b/pu_to_real & losses/eta_calc/0chk ==
  i : Inport
  Abs : Abs  SaturateOnIntegerOverflow=off
  MinMax1 : MinMax  Function=max  Inputs=2
  Switch3 : Switch  SaturateOnIntegerOverflow=off  InputSameDT=off
  V1 : Constant  Value=-1
  V3 : Constant
  n 2 : Constant  Value=1e-4
  x1 : Product  Inputs=**
  o : Outport
  wires:
  n 2/1 -> MinMax1/2
  Switch3/1 -> x1/1
  i/1 -> Switch3/2, Abs/1
  Abs/1 -> MinMax1/1
  x1/1 -> o/1
  V3/1 -> Switch3/1
  V1/1 -> Switch3/3
  MinMax1/1 -> x1/2

== system Porsche930Turbo_Model_V0/E-MOTOR/EM_model_v47b/pu_to_real & losses/eta_calc/0chk1 ==
  i : Inport
  Abs : Abs  SaturateOnIntegerOverflow=off
  MinMax1 : MinMax  Function=max  Inputs=2
  Switch3 : Switch  SaturateOnIntegerOverflow=off  InputSameDT=off
  V1 : Constant  Value=-1
  V3 : Constant
  n 2 : Constant  Value=1e-4
  x1 : Product  Inputs=**
  o : Outport
  wires:
  n 2/1 -> MinMax1/2
  Switch3/1 -> x1/1
  i/1 -> Switch3/2, Abs/1
  Abs/1 -> MinMax1/1
  x1/1 -> o/1
  V3/1 -> Switch3/1
  V1/1 -> Switch3/3
  MinMax1/1 -> x1/2

== system Porsche930Turbo_Model_V0/E-MOTOR/EM_model_v47b/pu_to_real & losses/eta_calc/0chk2 ==
  i : Inport
  Abs : Abs  SaturateOnIntegerOverflow=off
  MinMax1 : MinMax  Function=max  Inputs=2
  Switch3 : Switch  SaturateOnIntegerOverflow=off  InputSameDT=off
  V1 : Constant  Value=-1
  V3 : Constant
  n 2 : Constant  Value=1e-4
  x1 : Product  Inputs=**
  o : Outport
  wires:
  n 2/1 -> MinMax1/2
  Switch3/1 -> x1/1
  i/1 -> Switch3/2, Abs/1
  Abs/1 -> MinMax1/1
  x1/1 -> o/1
  V3/1 -> Switch3/1
  V1/1 -> Switch3/3
  MinMax1/1 -> x1/2

== system Porsche930Turbo_Model_V0/E-MOTOR/EM_model_v47b/pu_to_real & losses/mot+inv losses/DQmodule ==
  i : Inport
  Add : Sum
  Demux2 : Demux  Outputs=2
  Product : Product
  Product1 : Product
  Sqrt : Sqrt
  mod : Outport
  wires:
  Demux2/1 -> Product/2, Product/1
  Sqrt/1 -> mod/1
  Product/1 -> Add/1
  Demux2/2 -> Product1/1, Product1/2
  Add/1 -> Sqrt/1
  Product1/1 -> Add/2
  i/1 -> Demux2/1

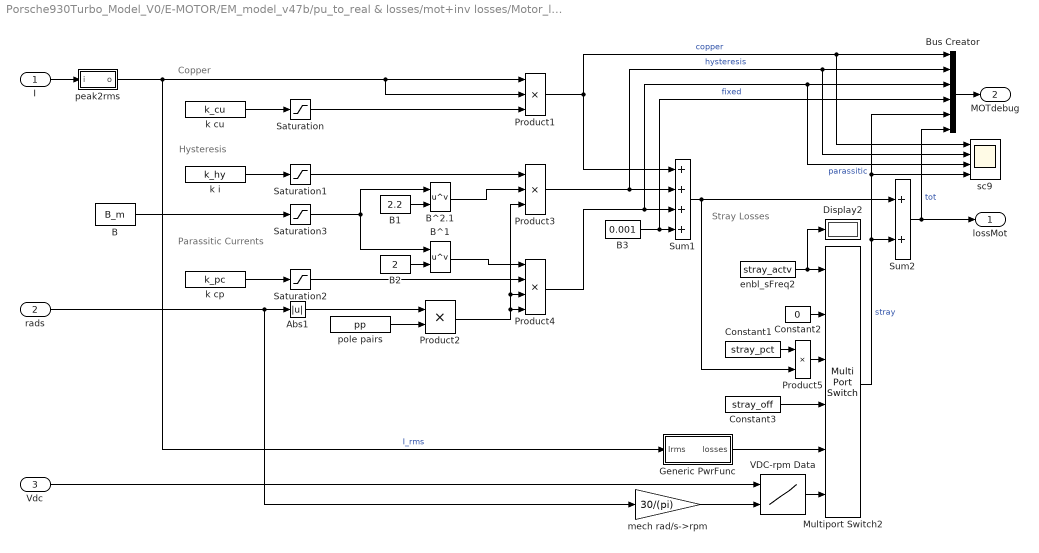
== system Porsche930Turbo_Model_V0/E-MOTOR/EM_model_v47b/pu_to_real & losses/mot+inv losses/Motor_losses ==
  note: Stray Losses
  note: Parassitic Currents
  note: Hysteresis
  note: Copper
  I : Inport
  rads : Inport  Port=2
  Vdc : Inport  Port=3
  Abs1 : Abs  SaturateOnIntegerOverflow=off
  B : Constant  Value=B_m
  B1 : Constant  Value=2.2
  B2 : Constant  Value=2
  B3 : Constant  Value=0.001
  B^1 : Math  Operator=pow
  B^2.1 : Math  Operator=pow
  Bus Creator : BusCreator  Inputs=6
  Constant1 : Constant  Value=stray_pct
  Constant2 : Constant  Value=0
  Constant3 : Constant  Value=stray_off
  Display2 : Display
  Generic PwrFunc : Subsystem
  Multiport Switch2 : MultiPortSwitch  Inputs=5  SaturateOnIntegerOverflow=off  InputSameDT=off
  Product1 : Product  Inputs=3
  Product2 : Product
  Product3 : Product  Inputs=3
  Product4 : Product  Inputs=4
  Product5 : Product
  Saturation{,1..3} (4 alike) : Saturate  UpperLimit=1e6  LowerLimit=0
  Sum1 : Sum  Inputs=++++
  Sum2 : Sum
  VDC-rpm Data : Lookup_n-D  BreakpointsForDimension1=stray_vdc  BreakpointsForDimension2=stray_rpm  BeginIndexSearchUsingPreviousIndexResult=on  Table=stray_watt  ExtrapMethod=Clip  UseLastTableValue=on  InternalRulePriority=Speed  RndMeth=Simplest
      settings: InputPortMap=u0,u1
  enbl_sFreq2 : Constant  Value=stray_actv
  k cp : Constant  Value=k_pc
  k cu : Constant  Value=k_cu
  k i : Constant  Value=k_hy
  mech rad/s->rpm : Gain  Gain=30/(pi)
  peak2rms : Subsystem
      mask Display: disp('pk2rms')
  pole pairs : Constant  Value=pp
  sc9 : Scope  NumInputPorts=4
      settings: DataLoggingVariableName=ScopeData5  DataLoggingSaveFormat=Array
  lossMot : Outport
  MOTdebug : Outport  Port=2
  wires:
  Product4/1 -> Bus Creator/3, sc9/3, Sum1/3  "parassitic"
  Product2/1 -> Product3/3, Product4/3, Product4/4
  B3/1 -> Bus Creator/4, Sum1/4  "fixed"
  Abs1/1 -> Product2/1
  I/1 -> peak2rms/1(i)
  k i/1 -> Saturation1/1
  pole pairs/1 -> Product2/2
  k cu/1 -> Saturation/1
  k cp/1 -> Saturation2/1
  Product3/1 -> Bus Creator/2, sc9/2, Sum1/2  "hysteresis"
  Product1/1 -> Bus Creator/1, sc9/1, Sum1/1  "copper"
  B^1/1 -> Product4/1
  B^2.1/1 -> Product3/2
  Sum1/1 -> Product5/2, Sum2/1
  Multiport Switch2/1 -> Bus Creator/5, sc9/4, Sum2/2  "stray"
  Constant3/1 -> Multiport Switch2/4
  Vdc/1 -> VDC-rpm Data/1
  Product5/1 -> Multiport Switch2/3
  Constant1/1 -> Product5/1
  Constant2/1 -> Multiport Switch2/2
  enbl_sFreq2/1 -> Display2/1, Multiport Switch2/1
  Generic PwrFunc/1(losses) -> Multiport Switch2/5
  VDC-rpm Data/1 -> Multiport Switch2/6
  mech rad/s->rpm/1 -> VDC-rpm Data/2
  rads/1 -> mech rad/s->rpm/1, Abs1/1
  Sum2/1 -> Bus Creator/6, lossMot/1  "tot"
  peak2rms/1(o) -> Generic PwrFunc/1(Irms), Product1/2, Product1/1  "I_rms"
  B1/1 -> B^2.1/2
  B2/1 -> B^1/2
  B/1 -> Saturation3/1
  Bus Creator/1 -> MOTdebug/1
  Saturation/1 -> Product1/3
  Saturation1/1 -> Product3/1
  Saturation2/1 -> Product4/2
  Saturation3/1 -> B^1/1, B^2.1/1

== system Porsche930Turbo_Model_V0/E-MOTOR/EM_model_v47b/pu_to_real & losses/mot+inv losses/peak2rms ==
  i : Inport
  1/sqrt(2) : Gain  Gain=0.707106781186547
  o : Outport
  wires:
  i/1 -> 1/sqrt(2)/1  "peak value"
  1/sqrt(2)/1 -> o/1  "RMS value"

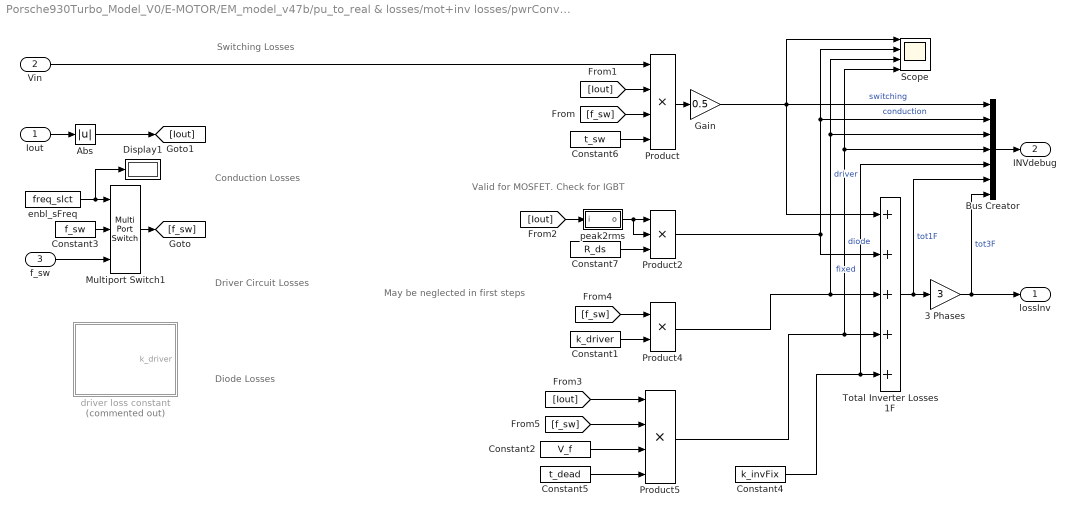
== system Porsche930Turbo_Model_V0/E-MOTOR/EM_model_v47b/pu_to_real & losses/mot+inv losses/pwrConv_losses ==
  note: Diode Losses
  note: Driver Circuit Losses
  note: Conduction Losses
  note: Switching Losses
  note: Valid for MOSFET. Check for IGBT
  note: May be neglected in first steps
  Iout : Inport
  Vin : Inport  Port=2
  f_sw : Inport  Port=3
  3 Phases : Gain  Gain=3
  Abs : Abs  SaturateOnIntegerOverflow=off
  Bus Creator : BusCreator  Inputs=7
  Constant1 : Constant  Value=k_driver
  Constant2 : Constant  Value=V_f
  Constant3 : Constant  Value=f_sw
  Constant4 : Constant  Value=k_invFix
  Constant5 : Constant  Value=t_dead
  Constant6 : Constant  Value=t_sw
  Constant7 : Constant  Value=R_ds
  Display1 : Display
  Gain : Gain  Gain=0.5
  Multiport Switch1 : MultiPortSwitch  Inputs=2  SaturateOnIntegerOverflow=off  InputSameDT=off
  Product : Product  Inputs=4
  Product2 : Product  Inputs=3
  Product4 : Product
  Product5 : Product  Inputs=4
  Scope : Scope  NumInputPorts=4
      settings: DataLoggingSaveFormat=Array
  Total Inverter Losses 1F : Sum  Inputs=+++++
  driver loss constant : Subsystem  Commented=on
  enbl_sFreq : Constant  Value=freq_slct
  peak2rms : Subsystem
      mask Display: disp('pk2rms')
  lossInv : Outport
  INVdebug : Outport  Port=2
  wires:
  Gain/1 -> Scope/1, Bus Creator/1, Total Inverter Losses 1F/1  "switching"
  Product5/1 -> Scope/4, Bus Creator/4, Total Inverter Losses 1F/4  "diode"
  Total Inverter Losses 1F/1 -> Bus Creator/6, 3 Phases/1  "tot1F"
  3 Phases/1 -> Bus Creator/7, lossInv/1  "tot3F"
  Product2/1 -> Scope/2, Bus Creator/2, Total Inverter Losses 1F/2  "conduction"
  Product4/1 -> Scope/3, Bus Creator/3, Total Inverter Losses 1F/3  "driver"
  Iout/1 -> Abs/1
  Product/1 -> Gain/1
  Vin/1 -> Product/1
  Constant6/1 -> Product/4
  Constant7/1 -> Product2/3
  Constant1/1 -> Product4/2
  Constant5/1 -> Product5/4
  [Iout] -> Product/2
  Constant2/1 -> Product5/3
  [f_sw] -> Product/3
  Abs/1 -> [Iout]
  [Iout] -> peak2rms/1(i)
  [Iout] -> Product5/1
  [f_sw] -> Product5/2
  [f_sw] -> Product4/1
  peak2rms/1(o) -> Product2/2, Product2/1
  Bus Creator/1 -> INVdebug/1
  enbl_sFreq/1 -> Display1/1, Multiport Switch1/1
  Constant3/1 -> Multiport Switch1/2
  Multiport Switch1/1 -> [f_sw]
  f_sw/1 -> Multiport Switch1/3
  Constant4/1 -> Bus Creator/5, Total Inverter Losses 1F/5  "fixed"

== system Porsche930Turbo_Model_V0/E-MOTOR/EM_model_v47b/pu_to_real & losses/output_mgmt/0chk1 ==
  i : Inport
  Abs : Abs  SaturateOnIntegerOverflow=off
  MinMax1 : MinMax  Function=max  Inputs=2
  Switch3 : Switch  SaturateOnIntegerOverflow=off  InputSameDT=off
  V1 : Constant  Value=-1
  V3 : Constant
  n 2 : Constant  Value=1e-4
  x1 : Product  Inputs=**
  o : Outport
  wires:
  n 2/1 -> MinMax1/2
  Switch3/1 -> x1/1
  i/1 -> Switch3/2, Abs/1
  Abs/1 -> MinMax1/1
  x1/1 -> o/1
  V3/1 -> Switch3/1
  V1/1 -> Switch3/3
  MinMax1/1 -> x1/2

== system Porsche930Turbo_Model_V0/E-MOTOR/EM_model_v47b/pu_to_real & losses/output_mgmt/0chk2 ==
  i : Inport
  Abs : Abs  SaturateOnIntegerOverflow=off
  MinMax1 : MinMax  Function=max  Inputs=2
  Switch3 : Switch  SaturateOnIntegerOverflow=off  InputSameDT=off
  V1 : Constant  Value=-1
  V3 : Constant
  n 2 : Constant  Value=1e-4
  x1 : Product  Inputs=**
  o : Outport
  wires:
  n 2/1 -> MinMax1/2
  Switch3/1 -> x1/1
  i/1 -> Switch3/2, Abs/1
  Abs/1 -> MinMax1/1
  x1/1 -> o/1
  V3/1 -> Switch3/1
  V1/1 -> Switch3/3
  MinMax1/1 -> x1/2

== system Porsche930Turbo_Model_V0/E-MOTOR/EM_model_v47b/pu_to_real & losses/trq_derating_TBD/0chk ==
  i : Inport
  Abs : Abs  SaturateOnIntegerOverflow=off
  MinMax1 : MinMax  Function=max  Inputs=2
  Switch3 : Switch  SaturateOnIntegerOverflow=off  InputSameDT=off
  V1 : Constant  Value=-1
  V3 : Constant
  n 2 : Constant  Value=1e-4
  x1 : Product  Inputs=**
  o : Outport
  wires:
  n 2/1 -> MinMax1/2
  Switch3/1 -> x1/1
  i/1 -> Switch3/2, Abs/1
  Abs/1 -> MinMax1/1
  x1/1 -> o/1
  V3/1 -> Switch3/1
  V1/1 -> Switch3/3
  MinMax1/1 -> x1/2

== system Porsche930Turbo_Model_V0/E-MOTOR/EM_model_v47b/pu_to_real & losses/trq_derating_TBD/0chk1 ==
  i : Inport
  Abs : Abs  SaturateOnIntegerOverflow=off
  MinMax1 : MinMax  Function=max  Inputs=2
  Switch3 : Switch  SaturateOnIntegerOverflow=off  InputSameDT=off
  V1 : Constant  Value=-1
  V3 : Constant
  n 2 : Constant  Value=1e-4
  x1 : Product  Inputs=**
  o : Outport
  wires:
  n 2/1 -> MinMax1/2
  Switch3/1 -> x1/1
  i/1 -> Switch3/2, Abs/1
  Abs/1 -> MinMax1/1
  x1/1 -> o/1
  V3/1 -> Switch3/1
  V1/1 -> Switch3/3
  MinMax1/1 -> x1/2

== system Porsche930Turbo_Model_V0/E-MOTOR/EM_model_v47b/pu_to_real & losses/trq_derating_TBD/0chk2 ==
  i : Inport
  Abs : Abs  SaturateOnIntegerOverflow=off
  MinMax1 : MinMax  Function=max  Inputs=2
  Switch3 : Switch  SaturateOnIntegerOverflow=off  InputSameDT=off
  V1 : Constant  Value=-1
  V3 : Constant
  n 2 : Constant  Value=1e-4
  x1 : Product  Inputs=**
  o : Outport
  wires:
  n 2/1 -> MinMax1/2
  Switch3/1 -> x1/1
  i/1 -> Switch3/2, Abs/1
  Abs/1 -> MinMax1/1
  x1/1 -> o/1
  V3/1 -> Switch3/1
  V1/1 -> Switch3/3
  MinMax1/1 -> x1/2

== system Porsche930Turbo_Model_V0/E-MOTOR/EM_model_v47b/pu_to_real & losses/trq_derating_TBD/DQmodule ==
  i : Inport
  Add : Sum
  Demux2 : Demux  Outputs=2
  Product : Product
  Product1 : Product
  Sqrt : Sqrt
  mod : Outport
  wires:
  Demux2/1 -> Product/2, Product/1
  Sqrt/1 -> mod/1
  Product/1 -> Add/1
  Demux2/2 -> Product1/1, Product1/2
  Add/1 -> Sqrt/1
  Product1/1 -> Add/2
  i/1 -> Demux2/1

== system Porsche930Turbo_Model_V0/E-MOTOR/EM_model_v47b/pu_to_real & losses/trq_derating_TBD/DQmodule1 ==
  i : Inport
  Add : Sum
  Demux2 : Demux  Outputs=2
  Product : Product
  Product1 : Product
  Sqrt : Sqrt
  mod : Outport
  wires:
  Demux2/1 -> Product/2, Product/1
  Sqrt/1 -> mod/1
  Product/1 -> Add/1
  Demux2/2 -> Product1/1, Product1/2
  Add/1 -> Sqrt/1
  Product1/1 -> Add/2
  i/1 -> Demux2/1

== system Porsche930Turbo_Model_V0/E-MOTOR/EM_model_v47b/pu_to_real & losses/trq_derating_TBD/DQmodule2 ==
  i : Inport
  Add : Sum
  Demux2 : Demux  Outputs=2
  Product : Product
  Product1 : Product
  Sqrt : Sqrt
  mod : Outport
  wires:
  Demux2/1 -> Product/2, Product/1
  Sqrt/1 -> mod/1
  Product/1 -> Add/1
  Demux2/2 -> Product1/1, Product1/2
  Add/1 -> Sqrt/1
  Product1/1 -> Add/2
  i/1 -> Demux2/1

== system Porsche930Turbo_Model_V0/E-MOTOR/EM_model_v47b/pu_to_real & losses/trq_derating_TBD/peak2rms ==
  i : Inport
  1/sqrt(2) : Gain  Gain=0.707106781186547
  o : Outport
  wires:
  i/1 -> 1/sqrt(2)/1  "peak value"
  1/sqrt(2)/1 -> o/1  "RMS value"

== system Porsche930Turbo_Model_V0/E-MOTOR/EM_model_v47b/pu_to_real & losses/trq_derating_TBD/peak2rms1 ==
  i : Inport
  1/sqrt(2) : Gain  Gain=0.707106781186547
  o : Outport
  wires:
  i/1 -> 1/sqrt(2)/1  "peak value"
  1/sqrt(2)/1 -> o/1  "RMS value"

== system Porsche930Turbo_Model_V0/E-MOTOR/EM_model_v47b/pu_to_real & losses/trq_derating_TBD/peak2rms2 ==
  i : Inport
  1/sqrt(2) : Gain  Gain=0.707106781186547
  o : Outport
  wires:
  i/1 -> 1/sqrt(2)/1  "peak value"
  1/sqrt(2)/1 -> o/1  "RMS value"

== system Porsche930Turbo_Model_V0/E-MOTOR/EM_model_v47b/Motor_Model/blockD/idq_max_MTC-I0/id_mtcMax ==
  I0 : Inport
  0chk : Subsystem
      mask Display: disp('0chk')
  Add1 : Sum
  Add2 : Sum
  Add3 : Sum  Inputs=-+
  Comp2Const1 : simulink/Logic and Bit Operations/Compare To Constant  relop=>  const=1  OutDataTypeStr=boolean
  Constant2 : Constant  Value=r1
  Constant3 : Constant  Value=a
  Constant4 : Constant  Value=r
  Display1 : Display
  Display2 : Display
  Display3 : Display
  Gain1 : Gain  Gain=8
  Gain4 : Gain  Gain=4
  Product{1,3,5..6} (4 alike) : Product
  Product4 : Product  Inputs=*/
  Sqrt : Sqrt
  Switch2 : Switch  Criteria=u2 > Threshold  SaturateOnIntegerOverflow=off  InputSameDT=off
  scope : Scope  NumInputPorts=2
      settings: DataLoggingVariableName=ScopeData5  DataLoggingSaveFormat=Array
  id_MTC : Outport
  wires:
  I0/1 -> Product1/1, Display3/1, scope/1, Product6/1
  Constant2/1 -> Product1/2
  Product1/1 -> Product3/1, Product3/2, Gain4/1
  Product3/1 -> Gain1/1
  Gain1/1 -> Add1/2
  Switch2/1 -> Product4/1
  Gain4/1 -> 0chk/1(i)
  Product5/1 -> Add1/1
  Add2/1 -> Switch2/1
  Sqrt/1 -> Add2/2, Add3/2
  Add3/1 -> Switch2/3
  Constant4/1 -> Display2/1, Comp2Const1/1
  Add1/1 -> Sqrt/1
  Comp2Const1/1 -> Switch2/2
  0chk/1(o) -> Product4/2
  Product6/1 -> scope/2, id_MTC/1
  Product4/1 -> Product6/2
  Constant3/1 -> Display1/1, Product5/2, Product5/1, Add3/1, Add2/1

== system Porsche930Turbo_Model_V0/E-MOTOR/EM_model_v47b/Motor_Model/blockD/idq_max_MTC-I0/iq_mtcMax ==
  IO : Inport
  id : Inport  Port=2
  0ck1 : Subsystem
      mask Display: text(0.5,0.5,'|x|','HorizontalAlignment','center')
  Add : Sum  Inputs=+-
  Product : Product
  Product1 : Product
  Sqrt : Sqrt
  iq : Outport
  wires:
  Sqrt/1 -> iq/1
  Product/1 -> Add/1
  Add/1 -> 0ck1/1(i)
  Product1/1 -> Add/2
  IO/1 -> Product/2, Product/1
  id/1 -> Product1/1, Product1/2
  0ck1/1(o) -> Sqrt/1

== system Porsche930Turbo_Model_V0/E-MOTOR/EM_model_v47b/Motor_Model/blockD/idq_max_MTC-I0/sign ==
  i : Inport
  Switch3 : Switch  SaturateOnIntegerOverflow=off  InputSameDT=off
  V1 : Constant  Value=-1
  V3 : Constant
  o : Outport
  wires:
  i/1 -> Switch3/2
  Switch3/1 -> o/1
  V3/1 -> Switch3/1
  V1/1 -> Switch3/3

== system Porsche930Turbo_Model_V0/E-MOTOR/EM_model_v47b/Motor_Model/limits_MaxMin/current limits calc/DQmodule ==
  i : Inport
  Add : Sum
  Demux2 : Demux  Outputs=2
  Product : Product
  Product1 : Product
  Sqrt : Sqrt
  mod : Outport
  wires:
  Demux2/1 -> Product/2, Product/1
  Sqrt/1 -> mod/1
  Product/1 -> Add/1
  Demux2/2 -> Product1/1, Product1/2
  Add/1 -> Sqrt/1
  Product1/1 -> Add/2
  i/1 -> Demux2/1

== system Porsche930Turbo_Model_V0/E-MOTOR/EM_model_v47b/Motor_Model/limits_MaxMin/current limits calc/DQmodule1 ==
  i : Inport
  Add : Sum
  Demux2 : Demux  Outputs=2
  Product : Product
  Product1 : Product
  Sqrt : Sqrt
  mod : Outport
  wires:
  Demux2/1 -> Product/2, Product/1
  Sqrt/1 -> mod/1
  Product/1 -> Add/1
  Demux2/2 -> Product1/1, Product1/2
  Add/1 -> Sqrt/1
  Product1/1 -> Add/2
  i/1 -> Demux2/1

== system Porsche930Turbo_Model_V0/E-MOTOR/EM_model_v47b/pu_to_real & losses/mot+inv losses/Motor_losses/Generic PwrFunc ==
  Irms : Inport
  Add1 : Sum  Inputs=+++
  Product6 : Product  Inputs=3
  Product7 : Product
  k s0 : Constant  Value=k_s0
  k s1 : Constant  Value=k_s1
  k s2 : Constant  Value=k_s2
  losses : Outport
  wires:
  Product7/1 -> Add1/2
  Product6/1 -> Add1/1
  k s2/1 -> Product6/3
  Irms/1 -> Product7/1, Product6/2, Product6/1
  k s0/1 -> Add1/3
  Add1/1 -> losses/1
  k s1/1 -> Product7/2

== system Porsche930Turbo_Model_V0/E-MOTOR/EM_model_v47b/pu_to_real & losses/mot+inv losses/Motor_losses/peak2rms ==
  i : Inport
  1/sqrt(2) : Gain  Gain=0.707106781186547
  o : Outport
  wires:
  i/1 -> 1/sqrt(2)/1  "peak value"
  1/sqrt(2)/1 -> o/1  "RMS value"

== system Porsche930Turbo_Model_V0/E-MOTOR/EM_model_v47b/pu_to_real & losses/mot+inv losses/pwrConv_losses/driver loss constant ==
  Add{,1..3} (4 alike) : Sum
  Constant10 : Constant  Value=R_gi
  Constant13 : Constant  Value=R_ghi
  Constant14 : Constant  Value=R_glo
  Constant15 : Constant  Value=R_g
  Constant8 : Constant  Value=V_drv
  Constant9 : Constant  Value=Q_gTot
  Divide : Product  Inputs=*/
  Divide1 : Product  Inputs=*/
  Gain1 : Gain  Gain=0.5
  Product1 : Product  Inputs=3
  k_driver : Outport
  wires:
  Add3/1 -> Product1/3
  Add/1 -> Add2/2, Add1/2
  Product1/1 -> Gain1/1
  Constant10/1 -> Add/2  "R_Gi"
  Gain1/1 -> k_driver/1
  Divide1/1 -> Add3/2
  Divide/1 -> Add3/1
  Constant13/1 -> Add2/1, Divide/1  "R_GHi"
  Add1/1 -> Divide1/2
  Add2/1 -> Divide/2
  Constant15/1 -> Add/1  "R_G"
  Constant14/1 -> Divide1/1, Add1/1  "R_GLo"
  Constant8/1 -> Product1/1
  Constant9/1 -> Product1/2

== system Porsche930Turbo_Model_V0/E-MOTOR/EM_model_v47b/pu_to_real & losses/mot+inv losses/pwrConv_losses/peak2rms ==
  i : Inport
  1/sqrt(2) : Gain  Gain=0.707106781186547
  o : Outport
  wires:
  i/1 -> 1/sqrt(2)/1  "peak value"
  1/sqrt(2)/1 -> o/1  "RMS value"

== system Porsche930Turbo_Model_V0/E-MOTOR/EM_model_v47b/Motor_Model/blockD/idq_max_MTC-I0/id_mtcMax/0chk ==
  i : Inport
  Abs : Abs  SaturateOnIntegerOverflow=off
  MinMax1 : MinMax  Function=max  Inputs=2
  Switch3 : Switch  SaturateOnIntegerOverflow=off  InputSameDT=off
  V1 : Constant  Value=-1
  V3 : Constant
  n 2 : Constant  Value=1e-4
  x1 : Product  Inputs=**
  o : Outport
  wires:
  n 2/1 -> MinMax1/2
  Switch3/1 -> x1/1
  i/1 -> Switch3/2, Abs/1
  Abs/1 -> MinMax1/1
  x1/1 -> o/1
  V3/1 -> Switch3/1
  V1/1 -> Switch3/3
  MinMax1/1 -> x1/2
